simulink model "FMS"  (R2018b)
settings: configuration reference "fms_config" (kept outside this file)
values from neighbouring files (symbols this model uses):
  FMS_EXPORT = Simulink.Parameter(FMS_EXPORT_VALUE)    [fms_model_init.m]
  FMS_PARAM = Simulink.Parameter(FMS_PARAM_VALUE)    [fms_model_init.m]
undefined symbols (not defined in the file or in its folder): actuator_cmd, ax_cmd, ay_cmd, az_cmd, cmd_mask, ControlMode, ctrl_mode, DiscIntNeverNeededParam, FMS_Cmd, FMS_CONST, FMS_Error, home, mode, p_cmd, phi_cmd, PilotMode, psi_rate_cmd, q_cmd, r_cmd, reset, state, status, theta_cmd, throttle_cmd, timestamp, u_cmd, v_cmd, VehicleState, VehicleStatus, w_cmd, wp_consume, wp_current
libraries: simulink x123, FMT_Model_Lib x62, hdlsllib x13
(part 2 of 7)

== system FMS/FMS Commander/Commander/Arm/SubMode/Land ==
  FMS_In : Inport
  Action Port : ActionPort  InitializeStates=reset  ActionType=case
      settings: CopyFcn=Stateflow.SLINSF.SimulinkMan.removeBlockPreDeleteFcn
  Assist Land Speed : Subsystem
  Bus Assignment1 : BusAssignment  AssignedSignals=status,state,ctrl_mode,psi_rate_cmd,u_cmd,v_cmd,w_cmd
  Bus Selector : BusSelector  OutputSignals=Cmd_In.sp_waypoint
  Constant : Constant  Value=0  OutDataTypeStr=Inherit: Inherit via back propagation
  Constant1 : Constant  Value=0  OutDataTypeStr=Bus: FMS_Out_Bus
  Constant2 : Constant  Value=ControlMode.POSCTL
  Constant3 : Constant  Value=VehicleState.Land
  Constant6 : Constant  Value=VehicleStatus.Arm
  Data Type Conversion : DataTypeConversion
  Data Type Conversion1 : DataTypeConversion
  Data Type Conversion2 : DataTypeConversion
  Position Command : Subsystem
  Selector : Selector  InputPortWidth=3  IndexOptions=Index vector (dialog)  Indices=[1 2]  OutputSizes=1
  FMS_Out : Outport
  wires:
  Selector/1 -> Position Command/2(land_xy_R)
  Bus Assignment1/1 -> FMS_Out/1
  Constant1/1 -> Bus Assignment1/1
  Position Command/1(u_cmd_mPs) -> Bus Assignment1/6
  Position Command/2(v_cmd_mPs) -> Bus Assignment1/7
  Constant/1 -> Bus Assignment1/5
  Constant2/1 -> Data Type Conversion2/1
  Constant6/1 -> Data Type Conversion/1
  Data Type Conversion/1 -> Bus Assignment1/2
  Constant3/1 -> Data Type Conversion1/1
  Data Type Conversion1/1 -> Bus Assignment1/3
  Data Type Conversion2/1 -> Bus Assignment1/4
  Bus Selector/1 -> Selector/1  "<sp_waypoint>"
  FMS_In/1 -> Assist Land Speed/1(FMS_In), Position Command/1(FMS_In), Bus Selector/1
  Assist Land Speed/1(w_cmd_mPs) -> Bus Assignment1/8

== system FMS/FMS Commander/Commander/Arm/SubMode/Return ==
  FMS_In : Inport
  Action Port : ActionPort  InitializeStates=reset  ActionType=case
      settings: CopyFcn=Stateflow.SLINSF.SimulinkMan.removeBlockPreDeleteFcn
  Bus Assignment1 : BusAssignment  AssignedSignals=status,state,ctrl_mode,u_cmd,v_cmd,w_cmd,psi_rate_cmd
  Constant1 : Constant  Value=VehicleState.Return
  Constant2 : Constant  Value=0  OutDataTypeStr=Bus: FMS_Out_Bus
  Constant3 : Constant  Value=ControlMode.POSCTL
  Constant6 : Constant  Value=VehicleStatus.Arm
  Data Type Conversion : DataTypeConversion
  Data Type Conversion1 : DataTypeConversion
  Data Type Conversion2 : DataTypeConversion
  Heading Commander : Subsystem
  Sum : Sum  Inputs=+-|
  Velocity Commander : Subsystem
  Way Points : Subsystem
  FMS_Out : Outport
  wires:
  Sum/1 -> Heading Commander/2(p1p2)
  Way Points/2(p2) -> Velocity Commander/2(p2), Sum/1
  Way Points/3(p3) -> Velocity Commander/3(p3)
  Constant3/1 -> Data Type Conversion2/1
  Way Points/1(p1) -> Velocity Commander/1(p1), Sum/2
  Constant2/1 -> Bus Assignment1/1
  Heading Commander/2(psi_rad_cmd) -> Bus Assignment1/8
  Bus Assignment1/1 -> FMS_Out/1
  Data Type Conversion/1 -> Bus Assignment1/2
  Constant6/1 -> Data Type Conversion/1
  Data Type Conversion1/1 -> Bus Assignment1/3
  Data Type Conversion2/1 -> Bus Assignment1/4
  Constant1/1 -> Data Type Conversion1/1
  FMS_In/1 -> Heading Commander/1(FMS_In), Velocity Commander/4(FMS_In), Way Points/1(FMS_In)
  Velocity Commander/1(u_cmd) -> Bus Assignment1/5
  Velocity Commander/2(v_cmd) -> Bus Assignment1/6
  Velocity Commander/3(w_cmd) -> Bus Assignment1/7
  Heading Commander/1(psi_err_rad) -> Velocity Commander/5(psi_err_rad)

== system FMS/FMS Commander/Commander/Arm/SubMode/Takeoff ==
  FMS_In : Inport
  Action Port : ActionPort  InitializeStates=reset  ActionType=case
      settings: CopyFcn=Stateflow.SLINSF.SimulinkMan.removeBlockPreDeleteFcn
  Bus Assignment1 : BusAssignment  AssignedSignals=status,state,ctrl_mode,psi_rate_cmd,u_cmd,v_cmd,w_cmd
  Climb Speed : Subsystem
  Constant : Constant  Value=0  OutDataTypeStr=Inherit: Inherit via back propagation
  Constant1 : Constant  Value=0  OutDataTypeStr=Bus: FMS_Out_Bus
  Constant2 : Constant  Value=ControlMode.POSCTL
  Constant3 : Constant  Value=VehicleState.Takeoff
  Constant5 : Constant  Value=VehicleStatus.Arm
  Data Type Conversion : DataTypeConversion
  Data Type Conversion1 : DataTypeConversion
  Data Type Conversion2 : DataTypeConversion
  Demux : Demux  Outputs=2
  Track Position : Subsystem
  FMS_Out : Outport
  wires:
  Constant5/1 -> Data Type Conversion/1
  Demux/2 -> Bus Assignment1/7
  Demux/1 -> Bus Assignment1/6
  Constant/1 -> Bus Assignment1/5
  Constant2/1 -> Data Type Conversion2/1
  Track Position/1(uv_cmd_mPs) -> Demux/1
  Constant1/1 -> Bus Assignment1/1
  FMS_In/1 -> Climb Speed/1(FMS_In), Track Position/1(FMS_In)
  Bus Assignment1/1 -> FMS_Out/1
  Data Type Conversion/1 -> Bus Assignment1/2
  Data Type Conversion1/1 -> Bus Assignment1/3
  Constant3/1 -> Data Type Conversion1/1
  Data Type Conversion2/1 -> Bus Assignment1/4
  Climb Speed/1(w_cmd_mPs) -> Bus Assignment1/8

== system FMS/FMS Commander/Commander/Arm/SubMode/Unknown ==
  Action Port : ActionPort  InitializeStates=reset  ActionType=default
  Bus Assignment : BusAssignment  AssignedSignals=reset,status,state,actuator_cmd
  Constant : Constant  Value=0  OutDataTypeStr=Bus: FMS_Out_Bus
  Constant1 : Constant  Value=VehicleStatus.Disarm
  Constant2 : Constant  OutDataTypeStr=Inherit: Inherit via back propagation
  Constant3 : Constant  Value=[1000;1000;1000;1000]  VectorParams1D=off  OutDataTypeStr=Inherit: Inherit via back propagation
  Constant4 : Constant  Value=zeros(12,1)  OutDataTypeStr=Inherit: Inherit via back propagation
  Constant5 : Constant  Value=VehicleState.Disarm
  Data Type Conversion : DataTypeConversion
  Data Type Conversion1 : DataTypeConversion
  Mux : Mux  Inputs=2
  FMS_Out : Outport
  wires:
  Mux/1 -> Bus Assignment/5
  Constant4/1 -> Mux/2
  Constant3/1 -> Mux/1
  Constant1/1 -> Data Type Conversion/1
  Constant2/1 -> Bus Assignment/2
  Bus Assignment/1 -> FMS_Out/1
  Constant/1 -> Bus Assignment/1
  Constant5/1 -> Data Type Conversion1/1
  Data Type Conversion/1 -> Bus Assignment/3
  Data Type Conversion1/1 -> Bus Assignment/4

== system FMS/FMS Commander/Commander/Arm/Assist/Acro/Angular Rate Command ==
  FMS_In : Inport
  Bus Selector : BusSelector  OutputSignals=Pilot_Cmd.stick_roll,Pilot_Cmd.stick_pitch,Pilot_Cmd.stick_yaw
  Gain : Gain  Gain=pi  OutDataTypeStr=single
  Gain1 : Gain  Gain=-pi  OutDataTypeStr=single
  Gain2 : Gain  Gain=pi/2  OutDataTypeStr=single
  p_cmd_radPs : Outport
  q_cmd_radPs : Outport  Port=2
  r_cmd_radPs : Outport  Port=3
  wires:
  FMS_In/1 -> Bus Selector/1
  Gain2/1 -> r_cmd_radPs/1
  Gain1/1 -> q_cmd_radPs/1
  Bus Selector/3 -> Gain2/1  "<stick_yaw>"
  Bus Selector/2 -> Gain1/1  "<stick_pitch>"
  Gain/1 -> p_cmd_radPs/1
  Bus Selector/1 -> Gain/1  "<stick_roll>"

== system FMS/FMS Commander/Commander/Arm/Assist/Acro/Throttle Command ==
  FMS_In : Inport
  Add : Sum
  Bus Selector : BusSelector  OutputSignals=Pilot_Cmd.stick_throttle
  Constant4 : Constant  OutDataTypeStr=single
  Constant5 : Constant  Value=1000  OutDataTypeStr=uint16
  Gain2 : Gain  Gain=500  OutDataTypeStr=uint16
  Saturation : Saturate  UpperLimit=2  LowerLimit=0
  Sum : Sum  Inputs=|++
  throttle_cmd : Outport
  wires:
  Constant4/1 -> Sum/2
  Add/1 -> throttle_cmd/1
  Constant5/1 -> Add/2
  Bus Selector/1 -> Sum/1  "<stick_throttle>"
  Saturation/1 -> Gain2/1
  Sum/1 -> Saturation/1
  Gain2/1 -> Add/1
  FMS_In/1 -> Bus Selector/1

== system FMS/FMS Commander/Commander/Arm/Assist/Altitude/Altitude Command ==
  FMS_In : Inport
  Bus Selector : BusSelector  OutputSignals=pilot_cmd_lost
  Constant : Constant  Value=0.5  OutDataTypeStr=single
  Controller : Subsystem
  Detect Movement : Subsystem
  Switch : Switch  Criteria=u2 > Threshold
  w_cmd_mPs : Outport
  wires:
  Controller/1(w_cmd_mPs) -> Switch/3
  Detect Movement/1(motion_state) -> Controller/1(motion_state)
  FMS_In/1 -> Bus Selector/1, Controller/2(FMS_In), Detect Movement/1(FMS_In)
  Bus Selector/1 -> Switch/2  "<pilot_cmd_lost>"
  Constant/1 -> Switch/1
  Switch/1 -> w_cmd_mPs/1

== system FMS/FMS Commander/Commander/Arm/Assist/Altitude/Attitude Command ==
  FMS_In : Inport
  Bus Selector : BusSelector  OutputSignals=Pilot_Cmd.stick_roll,Pilot_Cmd.stick_pitch
  Bus Selector1 : BusSelector  OutputSignals=pilot_cmd_lost
  Compare To Constant : simulink/Logic and Bit Operations/Compare To Constant  relop=>  const=1  OutDataTypeStr=boolean
  Data Type Conversion : DataTypeConversion  OutDataTypeStr=single
  DeadZone : Subsystem  mask{th=FMS_PARAM.MC_ROLL_DZ}
      mask prompts: th "Threshold"
      mask Display: disp('Dead Zone')
  DeadZone2 : Subsystem  mask{th=FMS_PARAM.MC_PITCH_DZ}
      mask prompts: th "Threshold"
      mask Display: disp('Dead Zone')
  Demux : Demux  Outputs=2
  Gain : Gain  Gain=FMS_PARAM.MC_ATT_LIM
  Gain1 : Gain  Gain=-FMS_PARAM.MC_ATT_LIM
  Logical Operator : Logic  Operator=NOT  AllPortsSameDT=off  OutDataTypeStr=boolean
  Multiply : Product
  Multiply1 : Product
  Mux : Mux  Inputs=2
  Phi_CMD_TD : Subsystem
  Switch : Switch  Criteria=u2 > Threshold
  Theta_CMD_TD : Subsystem
  Vector Modulus : FMT_Model_Lib/Math/Vector Modulus
      settings: SourceProductName=FMT Toolbox
  Vector Normalize : FMT_Model_Lib/Math/Vector Normalize
      settings: SourceProductName=FMT Toolbox
  phi_cmd_radPs : Outport
  theta_cmd_radPs : Outport  Port=2
  wires:
  Bus Selector/2 -> DeadZone2/1(u)  "<stick_pitch>"
  Bus Selector/1 -> DeadZone/1(u)  "<stick_roll>"
  FMS_In/1 -> Bus Selector1/1, Bus Selector/1
  Gain/1 -> Multiply/2
  Bus Selector1/1 -> Logical Operator/1  "<pilot_cmd_lost>"
  Multiply/1 -> Phi_CMD_TD/1(v)
  Gain1/1 -> Multiply1/2
  Multiply1/1 -> Theta_CMD_TD/1(v)
  Logical Operator/1 -> Data Type Conversion/1
  Data Type Conversion/1 -> Multiply1/1, Multiply/1
  DeadZone/1(y) -> Mux/1
  DeadZone2/1(y) -> Mux/2
  Mux/1 -> Switch/3, Vector Normalize/1, Vector Modulus/1
  Vector Modulus/1 -> Compare To Constant/1
  Compare To Constant/1 -> Switch/2
  Vector Normalize/1 -> Switch/1
  Switch/1 -> Demux/1
  Demux/1 -> Gain/1
  Demux/2 -> Gain1/1
  Phi_CMD_TD/1(v1) -> phi_cmd_radPs/1
  Theta_CMD_TD/1(v1) -> theta_cmd_radPs/1

== system FMS/FMS Commander/Commander/Arm/Assist/Altitude/Heading Command ==
  FMS_In : Inport
  Controller : Subsystem
  Detect Movement : Subsystem
  psi_rate_cmd_radPs : Outport
  wires:
  FMS_In/1 -> Detect Movement/1(FMS_In), Controller/2(FMS_In)
  Controller/1(psi_rate_cmd_radPs) -> psi_rate_cmd_radPs/1
  Detect Movement/1(motion_state) -> Controller/1(motion_state)

== system FMS/FMS Commander/Commander/Arm/Assist/Position/Altitude Command ==
  FMS_In : Inport
  Bus Selector : BusSelector  OutputSignals=pilot_cmd_lost
  Constant : Constant  Value=0.5  OutDataTypeStr=single
  Controller : Subsystem
  Detect Movement : Subsystem
  Switch : Switch  Criteria=u2 > Threshold
  w_cmd_mPs : Outport
  wires:
  Controller/1(w_cmd_mPs) -> Switch/3
  Detect Movement/1(motion_state) -> Controller/1(motion_state)
  FMS_In/1 -> Bus Selector/1, Controller/2(FMS_In), Detect Movement/1(FMS_In)
  Bus Selector/1 -> Switch/2  "<pilot_cmd_lost>"
  Constant/1 -> Switch/1
  Switch/1 -> w_cmd_mPs/1

== system FMS/FMS Commander/Commander/Arm/Assist/Position/Heading Command ==
  FMS_In : Inport
  Controller : Subsystem
  Detect Movement : Subsystem
  psi_rate_cmd_radPs : Outport
  wires:
  FMS_In/1 -> Detect Movement/1(FMS_In), Controller/2(FMS_In)
  Detect Movement/1(motion_state) -> Controller/1(motion_state)
  Controller/1(psi_rate_cmd_radPs) -> psi_rate_cmd_radPs/1

== system FMS/FMS Commander/Commander/Arm/Assist/Position/Position Command ==
  FMS_In : Inport
  Controller : Subsystem
  Demux : Demux  Outputs=2
  Detect Movement : Subsystem
  u_cmd_mPs : Outport
  v_cmd_mPs : Outport  Port=2
  wires:
  FMS_In/1 -> Controller/2(FMS_In), Detect Movement/1(FMS_In)
  Demux/2 -> v_cmd_mPs/1
  Demux/1 -> u_cmd_mPs/1
  Controller/1(uv_cmd_mPs) -> Demux/1
  Detect Movement/1(motion_state) -> Controller/1(motion_state)

== system FMS/FMS Commander/Commander/Arm/Assist/Stabilize/Attitude Command ==
  FMS_In : Inport
  Bus Selector : BusSelector  OutputSignals=Pilot_Cmd.stick_roll,Pilot_Cmd.stick_pitch
  Bus Selector1 : BusSelector  OutputSignals=pilot_cmd_lost
  Compare To Constant : simulink/Logic and Bit Operations/Compare To Constant  relop=>  const=1  OutDataTypeStr=boolean
  Data Type Conversion : DataTypeConversion  OutDataTypeStr=single
  DeadZone : Subsystem  mask{th=FMS_PARAM.MC_ROLL_DZ}
      mask prompts: th "Threshold"
      mask Display: disp('Dead Zone')
  DeadZone2 : Subsystem  mask{th=FMS_PARAM.MC_PITCH_DZ}
      mask prompts: th "Threshold"
      mask Display: disp('Dead Zone')
  Demux : Demux  Outputs=2
  Gain : Gain  Gain=FMS_PARAM.MC_ATT_LIM
  Gain1 : Gain  Gain=-FMS_PARAM.MC_ATT_LIM
  Logical Operator : Logic  Operator=NOT  AllPortsSameDT=off  OutDataTypeStr=boolean
  Multiply : Product
  Multiply1 : Product
  Mux : Mux  Inputs=2
  Phi_CMD_TD : Subsystem
  Switch : Switch  Criteria=u2 > Threshold
  Theta_CMD_TD : Subsystem
  Vector Modulus : FMT_Model_Lib/Math/Vector Modulus
      settings: SourceProductName=FMT Toolbox
  Vector Normalize : FMT_Model_Lib/Math/Vector Normalize
      settings: SourceProductName=FMT Toolbox
  phi_cmd_radPs : Outport
  theta_cmd_radPs : Outport  Port=2
  wires:
  Bus Selector/2 -> DeadZone2/1(u)  "<stick_pitch>"
  Bus Selector/1 -> DeadZone/1(u)  "<stick_roll>"
  FMS_In/1 -> Bus Selector1/1, Bus Selector/1
  Gain/1 -> Multiply/2
  Bus Selector1/1 -> Logical Operator/1  "<pilot_cmd_lost>"
  Multiply/1 -> Phi_CMD_TD/1(v)
  Gain1/1 -> Multiply1/2
  Multiply1/1 -> Theta_CMD_TD/1(v)
  Logical Operator/1 -> Data Type Conversion/1
  Data Type Conversion/1 -> Multiply1/1, Multiply/1
  DeadZone/1(y) -> Mux/1
  DeadZone2/1(y) -> Mux/2
  Mux/1 -> Switch/3, Vector Normalize/1, Vector Modulus/1
  Vector Modulus/1 -> Compare To Constant/1
  Compare To Constant/1 -> Switch/2
  Vector Normalize/1 -> Switch/1
  Switch/1 -> Demux/1
  Demux/1 -> Gain/1
  Demux/2 -> Gain1/1
  Phi_CMD_TD/1(v1) -> phi_cmd_radPs/1
  Theta_CMD_TD/1(v1) -> theta_cmd_radPs/1

== system FMS/FMS Commander/Commander/Arm/Assist/Stabilize/Heading Command ==
  FMS_In : Inport
  Controller : Subsystem
  Detect Movement : Subsystem
  psi_rate_cmd_radPs : Outport
  wires:
  FMS_In/1 -> Detect Movement/1(FMS_In), Controller/2(FMS_In)
  Controller/1(psi_rate_cmd_radPs) -> psi_rate_cmd_radPs/1
  Detect Movement/1(motion_state) -> Controller/1(motion_state)

== system FMS/FMS Commander/Commander/Arm/Assist/Stabilize/Throttle Command ==
  FMS_In : Inport
  Add : Sum
  Bus Selector : BusSelector  OutputSignals=Pilot_Cmd.stick_throttle
  Bus Selector1 : BusSelector  OutputSignals=pilot_cmd_lost
  Constant : Constant  Value=FMS_PARAM.MC_LAND_LOCK_THRO  OutDataTypeStr=uint16
  Constant4 : Constant  OutDataTypeStr=single
  Constant5 : Constant  Value=1000  OutDataTypeStr=uint16
  Gain2 : Gain  Gain=500  OutDataTypeStr=uint16
  Saturation : Saturate  UpperLimit=2  LowerLimit=0
  Sum : Sum  Inputs=|++
  Switch : Switch  Criteria=u2 > Threshold
  throttle_cmd : Outport
  wires:
  FMS_In/1 -> Bus Selector1/1, Bus Selector/1
  Gain2/1 -> Add/1
  Sum/1 -> Saturation/1
  Saturation/1 -> Gain2/1
  Bus Selector/1 -> Sum/1  "<stick_throttle>"
  Constant5/1 -> Add/2
  Add/1 -> Switch/3
  Constant4/1 -> Sum/2
  Bus Selector1/1 -> Switch/2  "<pilot_cmd_lost>"
  Switch/1 -> throttle_cmd/1
  Constant/1 -> Switch/1

== system FMS/FMS Commander/Commander/Arm/Auto/Mission/Mission_SubSystem ==
  FMS_In : Inport
  Reset : ResetPort  DisableCoverage=on
  Bus Assignment : BusAssignment  AssignedSignals=status,state,ctrl_mode,u_cmd,v_cmd,w_cmd,psi_rate_cmd
  Constant : Constant  Value=0  OutDataTypeStr=Bus: FMS_Out_Bus
  Constant1 : Constant  Value=VehicleStatus.Arm
  Constant2 : Constant  Value=VehicleState.Mission
  Constant3 : Constant  Value=ControlMode.POSCTL
  Data Type Conversion : DataTypeConversion
  Data Type Conversion1 : DataTypeConversion
  Data Type Conversion2 : DataTypeConversion
  Heading Commander : Subsystem
  Velocity Commander : Subsystem
  Way Points : Subsystem
  FMS_Out : Outport
  wires:
  Data Type Conversion1/1 -> Bus Assignment/3
  Way Points/2(p2) -> Velocity Commander/2(p2)
  Constant1/1 -> Data Type Conversion/1
  Heading Commander/2(psi_rad_cmd) -> Bus Assignment/8
  Data Type Conversion2/1 -> Bus Assignment/4
  Data Type Conversion/1 -> Bus Assignment/2
  Constant2/1 -> Data Type Conversion1/1
  Way Points/1(p1) -> Velocity Commander/1(p1)
  Way Points/3(p3) -> Velocity Commander/3(p3)
  Velocity Commander/2(v_cmd) -> Bus Assignment/6
  Heading Commander/1(psi_err_rad) -> Velocity Commander/5(psi_err_rad)
  Constant3/1 -> Data Type Conversion2/1
  Constant/1 -> Bus Assignment/1
  Velocity Commander/3(w_cmd) -> Bus Assignment/7
  FMS_In/1 -> Velocity Commander/4(FMS_In), Heading Commander/1(FMS_In), Way Points/1(FMS_In)
  Velocity Commander/1(u_cmd) -> Bus Assignment/5
  Bus Assignment/1 -> FMS_Out/1

== system FMS/FMS Commander/Commander/Arm/Auto/Offboard/Acc_Command ==
  FMS_In : Inport
  Accel_Command : Subsystem
  Body_FRD : Subsystem
  Bus Selector1 : BusSelector  OutputSignals=INS_Out.psi
  Bus Selector3 : BusSelector  OutputSignals=Auto_Cmd.frame
  Command_Mask : Subsystem
  Demux : Demux  Outputs=3
  Global_Local_NED : Subsystem
  Index Vector : MultiPortSwitch  DataPortOrder=Zero-based contiguous  Inputs=4  zeroidx=on
  Local_FRD : Subsystem
  Multiply : Product
  ax_C_cmd : Outport
  ay_C_cmd : Outport  Port=2
  az_C_cmd : Outport  Port=3
  wires:
  FMS_In/1 -> Bus Selector3/1, Bus Selector1/1, Accel_Command/1(FMS_In), Command_Mask/1(FMS_In)
  Bus Selector3/1 -> Index Vector/1  "<frame>"
  Command_Mask/1(acc_mask) -> Multiply/2
  Global_Local_NED/1(acc_cmd_C) -> Index Vector/3, Index Vector/2
  Local_FRD/1(acc_cmd_C) -> Index Vector/4
  Body_FRD/1(acc_cmd_C) -> Index Vector/5
  Multiply/1 -> Global_Local_NED/2(acc_cmd_O), Body_FRD/1(acc_cmd_B), Local_FRD/2(acc_cmd_R)
  Bus Selector1/1 -> Local_FRD/1(psi), Global_Local_NED/1(psi)  "<psi>"
  Index Vector/1 -> Demux/1
  Demux/1 -> ax_C_cmd/1
  Demux/2 -> ay_C_cmd/1
  Demux/3 -> az_C_cmd/1
  Accel_Command/1(accel_cmd) -> Multiply/1

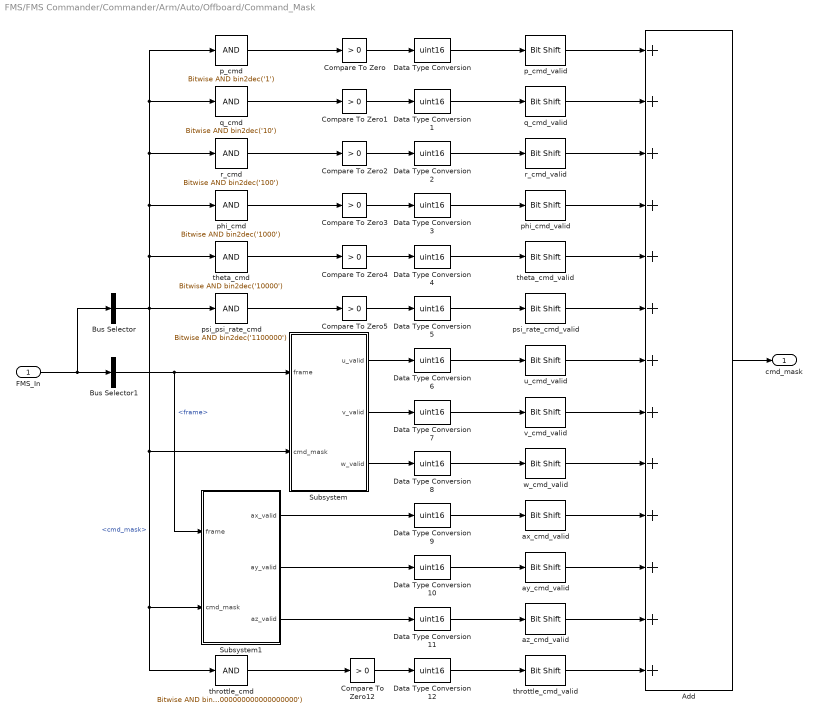
== system FMS/FMS Commander/Commander/Arm/Auto/Offboard/Command_Mask ==
  FMS_In : Inport
  Add : Sum  Inputs=+++++++++++++
  Bus Selector : BusSelector  OutputSignals=Auto_Cmd.cmd_mask
  Bus Selector1 : BusSelector  OutputSignals=Auto_Cmd.frame
  Compare To Zero{,1..5,12} (7 alike) : simulink/Logic and Bit Operations/Compare To Zero  relop=>  OutDataTypeStr=boolean
  Data Type Conversion{,1..12} (13 alike) : DataTypeConversion  OutDataTypeStr=uint16
  Subsystem : Subsystem
  Subsystem1 : Subsystem
  ax_cmd_valid : hdlsllib/Logic and Bit Operations/Bit Shift  mode=Shift Left Logical  N=9
      settings: SourceProductName=HDL Coder  SourceProductBaseCode=HD
  ay_cmd_valid : hdlsllib/Logic and Bit Operations/Bit Shift  mode=Shift Left Logical  N=10
      settings: SourceProductName=HDL Coder  SourceProductBaseCode=HD
  az_cmd_valid : hdlsllib/Logic and Bit Operations/Bit Shift  mode=Shift Left Logical  N=11
      settings: SourceProductName=HDL Coder  SourceProductBaseCode=HD
  p_cmd : simulink/Logic and Bit Operations/Bitwise Operator  logicop=AND  UseBitMask=on  BitMask=bin2dec('1')  BitMaskRealWorld=Stored Integer
  p_cmd_valid : hdlsllib/Logic and Bit Operations/Bit Shift  mode=Shift Left Logical  N=0
      settings: SourceProductName=HDL Coder  SourceProductBaseCode=HD
  phi_cmd : simulink/Logic and Bit Operations/Bitwise Operator  logicop=AND  UseBitMask=on  BitMask=bin2dec('1000')  BitMaskRealWorld=Stored Integer
  phi_cmd_valid : hdlsllib/Logic and Bit Operations/Bit Shift  mode=Shift Left Logical  N=3
      settings: SourceProductName=HDL Coder  SourceProductBaseCode=HD
  psi_psi_rate_cmd : simulink/Logic and Bit Operations/Bitwise Operator  logicop=AND  UseBitMask=on  BitMask=bin2dec('1100000')  BitMaskRealWorld=Stored Integer
  psi_rate_cmd_valid : hdlsllib/Logic and Bit Operations/Bit Shift  mode=Shift Left Logical  N=5
      settings: SourceProductName=HDL Coder  SourceProductBaseCode=HD
  q_cmd : simulink/Logic and Bit Operations/Bitwise Operator  logicop=AND  UseBitMask=on  BitMask=bin2dec('10')  BitMaskRealWorld=Stored Integer
  q_cmd_valid : hdlsllib/Logic and Bit Operations/Bit Shift  mode=Shift Left Logical  N=1
      settings: SourceProductName=HDL Coder  SourceProductBaseCode=HD
  r_cmd : simulink/Logic and Bit Operations/Bitwise Operator  logicop=AND  UseBitMask=on  BitMask=bin2dec('100')  BitMaskRealWorld=Stored Integer
  r_cmd_valid : hdlsllib/Logic and Bit Operations/Bit Shift  mode=Shift Left Logical  N=2
      settings: SourceProductName=HDL Coder  SourceProductBaseCode=HD
  theta_cmd : simulink/Logic and Bit Operations/Bitwise Operator  logicop=AND  UseBitMask=on  BitMask=bin2dec('10000')  BitMaskRealWorld=Stored Integer
  theta_cmd_valid : hdlsllib/Logic and Bit Operations/Bit Shift  mode=Shift Left Logical  N=4
      settings: SourceProductName=HDL Coder  SourceProductBaseCode=HD
  throttle_cmd : simulink/Logic and Bit Operations/Bitwise Operator  logicop=AND  UseBitMask=on  BitMask=bin2dec('10000000000000000000')  BitMaskRealWorld=Stored Integer
  throttle_cmd_valid : hdlsllib/Logic and Bit Operations/Bit Shift  mode=Shift Left Logical  N=12
      settings: SourceProductName=HDL Coder  SourceProductBaseCode=HD
  u_cmd_valid : hdlsllib/Logic and Bit Operations/Bit Shift  mode=Shift Left Logical  N=6
      settings: SourceProductName=HDL Coder  SourceProductBaseCode=HD
  v_cmd_valid : hdlsllib/Logic and Bit Operations/Bit Shift  mode=Shift Left Logical  N=7
      settings: SourceProductName=HDL Coder  SourceProductBaseCode=HD
  w_cmd_valid : hdlsllib/Logic and Bit Operations/Bit Shift  mode=Shift Left Logical  N=8
      settings: SourceProductName=HDL Coder  SourceProductBaseCode=HD
  cmd_mask : Outport
  wires:
  FMS_In/1 -> Bus Selector/1, Bus Selector1/1
  p_cmd/1 -> Compare To Zero/1
  Compare To Zero/1 -> Data Type Conversion/1
  Data Type Conversion/1 -> p_cmd_valid/1
  q_cmd/1 -> Compare To Zero1/1
  Compare To Zero1/1 -> Data Type Conversion1/1
  Data Type Conversion1/1 -> q_cmd_valid/1
  r_cmd/1 -> Compare To Zero2/1
  Compare To Zero2/1 -> Data Type Conversion2/1
  Data Type Conversion2/1 -> r_cmd_valid/1
  Data Type Conversion3/1 -> phi_cmd_valid/1
  phi_cmd/1 -> Compare To Zero3/1
  Compare To Zero3/1 -> Data Type Conversion3/1
  Data Type Conversion4/1 -> theta_cmd_valid/1
  theta_cmd/1 -> Compare To Zero4/1
  Compare To Zero4/1 -> Data Type Conversion4/1
  psi_psi_rate_cmd/1 -> Compare To Zero5/1
  Compare To Zero5/1 -> Data Type Conversion5/1
  Data Type Conversion5/1 -> psi_rate_cmd_valid/1
  Data Type Conversion9/1 -> ax_cmd_valid/1
  Bus Selector/1 -> q_cmd/1, p_cmd/1, r_cmd/1, phi_cmd/1, theta_cmd/1, throttle_cmd/1, Subsystem1/2(cmd_mask), Subsystem/2(cmd_mask), psi_psi_rate_cmd/1  "<cmd_mask>"
  Data Type Conversion10/1 -> ay_cmd_valid/1
  Data Type Conversion11/1 -> az_cmd_valid/1
  throttle_cmd/1 -> Compare To Zero12/1
  Compare To Zero12/1 -> Data Type Conversion12/1
  Data Type Conversion12/1 -> throttle_cmd_valid/1
  p_cmd_valid/1 -> Add/1
  q_cmd_valid/1 -> Add/2
  r_cmd_valid/1 -> Add/3
  phi_cmd_valid/1 -> Add/4
  theta_cmd_valid/1 -> Add/5
  psi_rate_cmd_valid/1 -> Add/6
  ax_cmd_valid/1 -> Add/10
  ay_cmd_valid/1 -> Add/11
  az_cmd_valid/1 -> Add/12
  throttle_cmd_valid/1 -> Add/13
  Add/1 -> cmd_mask/1
  u_cmd_valid/1 -> Add/7
  v_cmd_valid/1 -> Add/8
  w_cmd_valid/1 -> Add/9
  Data Type Conversion7/1 -> v_cmd_valid/1
  Data Type Conversion8/1 -> w_cmd_valid/1
  Data Type Conversion6/1 -> u_cmd_valid/1
  Subsystem/1(u_valid) -> Data Type Conversion6/1
  Subsystem/2(v_valid) -> Data Type Conversion7/1
  Subsystem/3(w_valid) -> Data Type Conversion8/1
  Bus Selector1/1 -> Subsystem/1(frame), Subsystem1/1(frame)  "<frame>"
  Subsystem1/1(ax_valid) -> Data Type Conversion9/1
  Subsystem1/2(ay_valid) -> Data Type Conversion10/1
  Subsystem1/3(az_valid) -> Data Type Conversion11/1

== system FMS/FMS Commander/Commander/Arm/Auto/Offboard/Heading_Command ==
  FMS_In : Inport
  Heading_Control : Subsystem
  Psi_Rate_Command : Subsystem
  Saturation : Saturate  UpperLimit=FMS_PARAM.MC_YAWRATE_LIM  LowerLimit=-FMS_PARAM.MC_YAWRATE_LIM
  Sum : Sum  Inputs=|++
  psi_rate_cmd : Outport
  wires:
  Sum/1 -> Saturation/1
  FMS_In/1 -> Heading_Control/1(FMS_In), Psi_Rate_Command/1(FMS_In)
  Heading_Control/1(psi_rate_cmd) -> Sum/1
  Psi_Rate_Command/1(psi_rate_cmd) -> Sum/2
  Saturation/1 -> psi_rate_cmd/1

== system FMS/FMS Commander/Commander/Arm/Auto/Offboard/Velocity_Command ==
  FMS_In : Inport
  Demux : Demux  Outputs=3
  Position_Control : Subsystem
  Saturation1 : Saturate  UpperLimit=FMS_PARAM.MC_VEL_XY_LIM  LowerLimit=-FMS_PARAM.MC_VEL_XY_LIM
  Saturation2 : Saturate  UpperLimit=FMS_PARAM.MC_VEL_XY_LIM  LowerLimit=-FMS_PARAM.MC_VEL_XY_LIM
  Saturation3 : Saturate  UpperLimit=FMS_PARAM.MC_VEL_Z_LIM  LowerLimit=-FMS_PARAM.MC_VEL_Z_LIM
  Sum1 : Sum  Inputs=|++
  Velocity_Command : Subsystem
  u_cmd : Outport
  v_cmd : Outport  Port=2
  w_cmd : Outport  Port=3
  wires:
  FMS_In/1 -> Velocity_Command/1(FMS_In), Position_Control/1(FMS_In)
  Position_Control/1(vel_cmd_C) -> Sum1/1
  Velocity_Command/1(vel_cmd_C) -> Sum1/2
  Demux/1 -> Saturation2/1
  Demux/2 -> Saturation1/1
  Demux/3 -> Saturation3/1
  Sum1/1 -> Demux/1
  Saturation2/1 -> u_cmd/1
  Saturation1/1 -> v_cmd/1
  Saturation3/1 -> w_cmd/1

== system FMS/FMS Commander/Commander/Arm/SubMode/Hold/Altitude Hold ==
  FMS_In : Inport
  Controller : Subsystem
  Detect Movement : Subsystem
  w_cmd_mPs : Outport
  wires:
  Controller/1(w_cmd_mPs) -> w_cmd_mPs/1
  Detect Movement/1(motion_state) -> Controller/1(motion_state)
  FMS_In/1 -> Controller/2(FMS_In), Detect Movement/1(FMS_In)

== system FMS/FMS Commander/Commander/Arm/SubMode/Hold/Heading Hold ==
  FMS_In : Inport
  Controller : Subsystem
  Detect Movement : Subsystem
  psi_rate_cmd_radPs : Outport
  wires:
  Controller/1(psi_rate_cmd_radPs) -> psi_rate_cmd_radPs/1
  Detect Movement/1(motion_state) -> Controller/1(motion_state)
  FMS_In/1 -> Controller/2(FMS_In), Detect Movement/1(FMS_In)

== system FMS/FMS Commander/Commander/Arm/SubMode/Hold/Position Hold ==
  FMS_In : Inport
  Controller : Subsystem
  Demux : Demux  Outputs=2
  Detect Movement : Subsystem
  u_cmd_mPs : Outport
  v_cmd_mPs : Outport  Port=2
  wires:
  FMS_In/1 -> Controller/2(FMS_In), Detect Movement/1(FMS_In)
  Demux/2 -> v_cmd_mPs/1
  Demux/1 -> u_cmd_mPs/1
  Controller/1(uv_cmd_mPs) -> Demux/1
  Detect Movement/1(motion_state) -> Controller/1(motion_state)

== system FMS/FMS Commander/Commander/Arm/SubMode/Land/Assist Land Speed ==
  FMS_In : Inport
  Bus Selector1 : BusSelector  OutputSignals=INS_Out.flag,INS_Out.h_AGL
  Compare To Constant : simulink/Logic and Bit Operations/Compare To Constant  relop=<=  const=FMS_PARAM.MC_ASSIST_LAND_H  OutDataTypeStr=boolean
  Gain : Gain  Gain=0.5
  Land_Speed : Constant  Value=FMS_PARAM.MC_LAND_SPEED  OutDataTypeStr=Inherit: Inherit via back propagation
  Logical Operator : Logic  AllPortsSameDT=off  OutDataTypeStr=boolean
  Switch : Switch  Criteria=u2 > Threshold
  TD : Subsystem
  cmd_p valid : simulink/Logic and Bit Operations/Bitwise Operator  logicop=AND  UseBitMask=on  BitMask=bin2dec('100000000')  BitMaskRealWorld=Stored Integer
  w_cmd_mPs : Outport
  wires:
  Land_Speed/1 -> Switch/3, Gain/1
  Gain/1 -> Switch/1
  Compare To Constant/1 -> Logical Operator/2
  FMS_In/1 -> Bus Selector1/1
  cmd_p valid/1 -> Logical Operator/1  "h_AGL_valid"
  Bus Selector1/1 -> cmd_p valid/1  "<flag>"
  Bus Selector1/2 -> Compare To Constant/1  "<h_AGL>"
  Logical Operator/1 -> Switch/2
  Switch/1 -> TD/1(v)
  TD/1(v1) -> w_cmd_mPs/1

== system FMS/FMS Commander/Commander/Arm/SubMode/Land/Position Command ==
  FMS_In : Inport
  land_xy_R : Inport  Port=2
  Demux : Demux  Outputs=2
  Position Control : Subsystem
  Saturation1 : Saturate  UpperLimit=FMS_PARAM.MC_VEL_XY_LIM/5  LowerLimit=-FMS_PARAM.MC_VEL_XY_LIM/5
  u_cmd_mPs : Outport
  v_cmd_mPs : Outport  Port=2
  wires:
  land_xy_R/1 -> Position Control/2(land_xy_R)
  Position Control/1(uv_cmd_mPs) -> Saturation1/1
  Demux/2 -> v_cmd_mPs/1
  Demux/1 -> u_cmd_mPs/1
  Saturation1/1 -> Demux/1
  FMS_In/1 -> Position Control/1(FMS_In)

== system FMS/FMS Commander/Commander/Arm/SubMode/Return/Heading Commander ==
  FMS_In : Inport
  p1p2 : Inport  Port=2
  Heading Control : Subsystem
  Included Angle : Subsystem
  North : Constant  Value=[1 0]  OutDataTypeStr=single
  psi_err_rad : Outport
  psi_rad_cmd : Outport  Port=2
  wires:
  p1p2/1 -> Included Angle/2(vec2)
  FMS_In/1 -> Heading Control/1(FMS_In)
  North/1 -> Included Angle/1(vec1)
  Included Angle/1(angle_rad) -> Heading Control/2(psi_cmd_rad)
  Heading Control/1(psi_rate_cmd_radPs) -> psi_rad_cmd/1
  Heading Control/2(psi_err_rad) -> psi_err_rad/1

== system FMS/FMS Commander/Commander/Arm/SubMode/Return/Velocity Commander ==
  p1 : Inport
  p2 : Inport  Port=2
  p3 : Inport  Port=3
  In Bus Element3 : Inport  Port=4  PortName=FMS_In
  In Bus Element4 : Inport  Port=4  PortName=FMS_In
  In Bus Element : Inport  Port=4  PortName=FMS_In  Element=INS_Out.vn
  In Bus Element1 : Inport  Port=4  PortName=FMS_In  Element=INS_Out.ve
  In Bus Element2 : Inport  Port=4  PortName=FMS_In  Element=INS_Out.psi
  In Bus Element5 : Inport  Port=4  PortName=FMS_In  Element=Cmd_In.set_speed
  psi_err_rad : Inport  Port=5
  Abs : Abs
  Altitude Control : Subsystem
  Compare To Constant : simulink/Logic and Bit Operations/Compare To Constant  relop=<=  const=10/180*pi  OutDataTypeStr=boolean
  Compare To Zero : simulink/Logic and Bit Operations/Compare To Zero  relop===  OutDataTypeStr=boolean
  Cruise Speed : Subsystem
  Demux : Demux  Outputs=3
  Gain : Gain  Gain=FMS_PARAM.MC_L1_GAIN  OutDataTypeStr=single
  Hold Position : Subsystem
  L1 Reference WP : Subsystem
  Lateral Acceleration : Subsystem
  Lateral Acceleration To Speed : Subsystem
  Mux1 : Mux  Inputs=2
  Switch : Switch  Criteria=u2 > Threshold
  "Target Speed " : Subsystem
  ValidCounter : Subsystem
  u_cmd : Outport
  v_cmd : Outport  Port=2
  w_cmd : Outport  Port=3
  wires:
  p3/1 -> "Target Speed "/1(P3), Lateral Acceleration To Speed/2(p3), Lateral Acceleration/3(p3), L1 Reference WP/3(P3)
  In Bus Element1/1 -> Mux1/2
  Mux1/1 -> Lateral Acceleration/1(Vg)
  p2/1 -> "Target Speed "/2(P2), Lateral Acceleration To Speed/3(p2), L1 Reference WP/2(P2)
  Demux/2 -> v_cmd/1
  Demux/3 -> w_cmd/1
  Demux/1 -> u_cmd/1
  In Bus Element/1 -> Mux1/1
  L1 Reference WP/1(L1_WP) -> Lateral Acceleration/2(L1_WP)  "L1_WP"
  p1/1 -> L1 Reference WP/1(P1)
  Lateral Acceleration/1(l1_a_cmd) -> Lateral Acceleration To Speed/1(l1_a)  "l1_a_cmd"
  In Bus Element2/1 -> Lateral Acceleration To Speed/4(psi)
  "Target Speed "/1(Vg) -> Lateral Acceleration To Speed/5(Vg)  "Vg"
  Lateral Acceleration To Speed/1(Vg_C_cmd) -> Altitude Control/2(Vg_C_cmd)
  psi_err_rad/1 -> Abs/1
  Abs/1 -> Compare To Constant/1
  In Bus Element3/1 -> Hold Position/1(FMS_In)
  Hold Position/1(vel_cmd) -> Switch/1
  Switch/1 -> Demux/1
  Altitude Control/1(vel_C_cmd) -> Switch/3
  In Bus Element4/1 -> Altitude Control/1(FMS_In)
  Compare To Constant/1 -> ValidCounter/1(in)
  ValidCounter/1(out) -> Compare To Zero/1
  Compare To Zero/1 -> Lateral Acceleration To Speed/7(rotating), "Target Speed "/4(rotating), Switch/2
  Cruise Speed/1(cruise_speed) -> Gain/1, Lateral Acceleration To Speed/6(cruise_speed), "Target Speed "/3(cruise_speed)
  In Bus Element5/1 -> Cruise Speed/1(config_speed)
  Gain/1 -> L1 Reference WP/4(L1), Lateral Acceleration/4(L1)

== system FMS/FMS Commander/Commander/Arm/SubMode/Return/Way Points ==
  note: P1: path start point
      | P2: path end point
      | P3: vehicle point
  FMS_In : Inport
  Bus Selector : BusSelector  OutputSignals=INS_Out.x_R,INS_Out.y_R
  Bus Selector1 : BusSelector  OutputSignals=Cmd_In.sp_waypoint
  Delay : Delay  DelayLength=1  InitialConditionSource=Input port  InitialCondition=single([0 0])
      settings: InputPortMap=u0,p4
  Mux : Mux  Inputs=2
  Reshape : Reshape  OutputDimensionality=Customize  OutputDimensions=[2,1]
  Reshape1 : Reshape  OutputDimensionality=Customize  OutputDimensions=[2,1]
  Reshape2 : Reshape  OutputDimensionality=Customize  OutputDimensions=[2,1]
  Selector : Selector  InputPortWidth=3  IndexOptions=Index vector (dialog)  Indices=[1 2]  OutputSizes=1
  p1 : Outport
  p2 : Outport  Port=2
  p3 : Outport  Port=3
  wires:
  Reshape2/1 -> p3/1
  Reshape1/1 -> p1/1
  Reshape/1 -> p2/1
  Bus Selector/2 -> Mux/2  "<y_R>"
  Bus Selector/1 -> Mux/1  "<x_R>"
  Mux/1 -> Reshape2/1, Delay/2
  Delay/1 -> Delay/1, Reshape1/1
  FMS_In/1 -> Bus Selector1/1, Bus Selector/1
  Bus Selector1/1 -> Selector/1  "<sp_waypoint>"
  Selector/1 -> Reshape/1

== system FMS/FMS Commander/Commander/Arm/SubMode/Takeoff/Climb Speed ==
  FMS_In : Inport
  Abs : Abs
  Abs1 : Abs
  Bus Selector : BusSelector  OutputSignals=INS_Out.h_R
  Bus Selector1 : BusSelector  OutputSignals=Cmd_In.cur_waypoint
  Bus Selector2 : BusSelector  OutputSignals=Cmd_In.sp_waypoint
  Compare To Constant : simulink/Logic and Bit Operations/Compare To Constant  relop=>  const=2.0  OutDataTypeStr=boolean
  Compare To Constant1 : simulink/Logic and Bit Operations/Compare To Constant  relop=>  const=2.0  OutDataTypeStr=boolean
  Gain : Gain  Gain=0.5
  Logical Operator : Logic  AllPortsSameDT=off  OutDataTypeStr=boolean
  Selector : Selector  InputPortWidth=3  IndexOptions=Index vector (dialog)  Indices=3  OutputSizes=1
  Selector1 : Selector  InputPortWidth=3  IndexOptions=Index vector (dialog)  Indices=3  OutputSizes=1
  Sum : Sum  Inputs=|+-
  Sum1 : Sum  Inputs=|+-
  Switch : Switch  Criteria=u2 ~= 0  Threshold=2
  TD : Subsystem
  Takeoff_Speed : Constant  Value=-FMS_PARAM.MC_TAKEOFF_SPEED  OutDataTypeStr=Inherit: Inherit via back propagation
  w_cmd_mPs : Outport
  wires:
  Takeoff_Speed/1 -> Gain/1, Switch/1
  Sum/1 -> Abs/1
  Bus Selector/1 -> Sum1/2, Sum/1  "<h_R>"
  Switch/1 -> TD/1(v)
  FMS_In/1 -> Bus Selector2/1, Bus Selector/1, Bus Selector1/1
  Selector/1 -> Sum/2
  Bus Selector1/1 -> Selector/1  "<cur_waypoint>"
  Abs/1 -> Compare To Constant1/1
  Bus Selector2/1 -> Selector1/1  "<sp_waypoint>"
  Selector1/1 -> Sum1/1
  Sum1/1 -> Abs1/1
  Abs1/1 -> Compare To Constant/1
  Compare To Constant/1 -> Logical Operator/1
  Compare To Constant1/1 -> Logical Operator/2
  Logical Operator/1 -> Switch/2
  TD/1(v1) -> w_cmd_mPs/1
  Gain/1 -> Switch/3

== system FMS/FMS Commander/Commander/Arm/SubMode/Takeoff/Track Position ==
  FMS_In : Inport
  Bus Selector : BusSelector  OutputSignals=INS_Out.psi
  Bus_Selection : Subsystem
  Constant : Constant  Value=0  OutDataTypeStr=Inherit: Inherit via back propagation
  Gain2 : Gain  Gain=FMS_PARAM.MC_XY_P  OutDataTypeStr=single
  Multiply : Product  Multiplication=Matrix(*)
  Mux : Mux  Inputs=2
  Psi To DCM : FMT_Model_Lib/Transformation/Psi To DCM
      settings: SourceProductName=FMT Toolbox
  Saturation1 : Saturate  UpperLimit=FMS_PARAM.MC_VEL_XY_LIM/5  LowerLimit=-FMS_PARAM.MC_VEL_XY_LIM/5
  Selector : Selector  InputPortWidth=3  IndexOptions=Index vector (dialog)  Indices=[1 2]  OutputSizes=1
  Sum : Sum  Inputs=-+|
  Target Position : Subsystem
  uv_cmd_mPs : Outport
  wires:
  Saturation1/1 -> uv_cmd_mPs/1
  Bus Selector/1 -> Psi To DCM/1  "<psi>"
  Selector/1 -> Gain2/1
  Mux/1 -> Multiply/2
  Multiply/1 -> Selector/1
  Psi To DCM/1 -> Multiply/1  "M_CO"
  Constant/1 -> Mux/2
  FMS_In/1 -> Bus Selector/1, Target Position/1(FMS_In), Bus_Selection/1(FMS_In)
  Sum/1 -> Mux/1  "xy_err_R"
  Bus_Selection/1(xy_est_R) -> Sum/1  "xy_est_R"
  Gain2/1 -> Saturation1/1
  Target Position/1(xy_cmd_R) -> Sum/2

== system FMS/FMS Commander/Commander/Arm/Assist/Altitude/Altitude Command/Controller ==
  motion_state : Inport
  In Bus Element : Inport  Port=2  PortName=FMS_In
  In Bus Element1 : Inport  Port=2  PortName=FMS_In
  Hold Control : Subsystem  TreatAsAtomicUnit=on
  Merge : Merge
  Move Control : Subsystem  TreatAsAtomicUnit=on
  Saturation1 : Saturate  UpperLimit=FMS_PARAM.MC_VEL_Z_LIM  LowerLimit=-FMS_PARAM.MC_VEL_Z_LIM
  Switch Case : SwitchCase  CaseConditions={MotionState.Hold, [MotionState.Brake, MotionState.Move]}  ShowDefaultCase=off
  w_cmd_mPs : Outport
  wires:
  Move Control/1(w_cmd_mPs) -> Merge/2
  Hold Control/1(w_cmd_mPs) -> Merge/1
  In Bus Element/1 -> Hold Control/1(FMS_In)
  Switch Case/1 -> Hold Control/Action
  motion_state/1 -> Switch Case/1
  Saturation1/1 -> w_cmd_mPs/1
  Merge/1 -> Saturation1/1
  Switch Case/2 -> Move Control/Action
  In Bus Element1/1 -> Move Control/1(FMS_In)

== system FMS/FMS Commander/Commander/Arm/Assist/Altitude/Altitude Command/Detect Movement ==
  FMS_In : Inport
  Abs : Abs
  Abs1 : Abs
  Bus Selector : BusSelector  OutputSignals=Pilot_Cmd.stick_throttle,INS_Out.vd
  Compare To Constant : simulink/Logic and Bit Operations/Compare To Constant  relop=>  const=FMS_PARAM.MC_THROTTLE_DZ  OutDataTypeStr=boolean
  Motion Status : Stateflow chart  TreatAsAtomicUnit=on
  motion_state : Outport
  wires:
  FMS_In/1 -> Bus Selector/1
  Abs1/1 -> Compare To Constant/1
  Motion Status/1(state) -> motion_state/1
  Compare To Constant/1 -> Motion Status/1(motion_req)
  Abs/1 -> Motion Status/2(speed)
  Bus Selector/1 -> Abs1/1  "<stick_throttle>"
  Bus Selector/2 -> Abs/1  "<vd>"

== system FMS/FMS Commander/Commander/Arm/Assist/Altitude/Attitude Command/DeadZone ==
  u : Inport
  Dead Zone : DeadZone  LowerValue=-th  UpperValue=th  SaturateOnIntegerOverflow=on
  Gain : Gain  Gain=1/(1-th)
  y : Outport
  wires:
  Gain/1 -> y/1
  Dead Zone/1 -> Gain/1
  u/1 -> Dead Zone/1

== system FMS/FMS Commander/Commander/Arm/Assist/Altitude/Attitude Command/DeadZone2 ==
  u : Inport
  Dead Zone : DeadZone  LowerValue=-th  UpperValue=th  SaturateOnIntegerOverflow=on
  Gain : Gain  Gain=1/(1-th)
  y : Outport
  wires:
  u/1 -> Dead Zone/1
  Dead Zone/1 -> Gain/1
  Gain/1 -> y/1

== system FMS/FMS Commander/Commander/Arm/Assist/Altitude/Attitude Command/Phi_CMD_TD ==
  v : Inport
  Constant : Constant  Value=FMS_PARAM.MC_STICK_SENS
  Integrator : DiscreteIntegrator  SampleTime=-1  ICPrevOutput=DiscIntNeverNeededParam  ICPrevScaledInput=DiscIntNeverNeededParam
  Integrator1 : DiscreteIntegrator  SampleTime=-1  ICPrevOutput=DiscIntNeverNeededParam  ICPrevScaledInput=DiscIntNeverNeededParam
  Subtract : Sum  Inputs=+-
  "fhan " : Subsystem  mask{r0=10*pi, h0=0.04}
      mask DialogControl ParameterGroupVar Prompt: fhan(v1,v2,r0,h0)
  v1 : Outport
  wires:
  "fhan "/1(fhan) -> Integrator/1
  Subtract/1 -> "fhan "/1(v1)
  Integrator/1 -> Integrator1/1, "fhan "/2(v2)  "v2"
  v/1 -> Subtract/2
  Integrator1/1 -> Subtract/1, v1/1
  Constant/1 -> "fhan "/3(scale)

== system FMS/FMS Commander/Commander/Arm/Assist/Altitude/Attitude Command/Theta_CMD_TD ==
  v : Inport
  Constant : Constant  Value=FMS_PARAM.MC_STICK_SENS
  Integrator : DiscreteIntegrator  SampleTime=-1  ICPrevOutput=DiscIntNeverNeededParam  ICPrevScaledInput=DiscIntNeverNeededParam
  Integrator1 : DiscreteIntegrator  SampleTime=-1  ICPrevOutput=DiscIntNeverNeededParam  ICPrevScaledInput=DiscIntNeverNeededParam
  Subtract : Sum  Inputs=+-
  "fhan " : Subsystem  mask{r0=10*pi, h0=0.04}
      mask DialogControl ParameterGroupVar Prompt: fhan(v1,v2,r0,h0)
  v1 : Outport
  wires:
  Integrator1/1 -> v1/1, Subtract/1
  v/1 -> Subtract/2
  Integrator/1 -> Integrator1/1, "fhan "/2(v2)  "v2"
  Subtract/1 -> "fhan "/1(v1)
  "fhan "/1(fhan) -> Integrator/1
  Constant/1 -> "fhan "/3(scale)

== system FMS/FMS Commander/Commander/Arm/Assist/Altitude/Heading Command/Controller ==
  motion_state : Inport
  In Bus Element : Inport  Port=2  PortName=FMS_In
  In Bus Element1 : Inport  Port=2  PortName=FMS_In
  Hold Control : Subsystem  TreatAsAtomicUnit=on
  Merge : Merge
  Move Control : Subsystem  TreatAsAtomicUnit=on
  Saturation : Saturate  UpperLimit=FMS_PARAM.MC_YAWRATE_LIM  LowerLimit=-FMS_PARAM.MC_YAWRATE_LIM
  Switch Case : SwitchCase  CaseConditions={MotionState.Hold, [MotionState.Brake, MotionState.Move]}  ShowDefaultCase=off
  psi_rate_cmd_radPs : Outport
  wires:
  Move Control/1(psi_rate_cmd_radPs) -> Merge/2
  Hold Control/1(psi_rate_cmd_radPs) -> Merge/1
  In Bus Element/1 -> Hold Control/1(FMS_In)
  Switch Case/2 -> Move Control/Action
  Switch Case/1 -> Hold Control/Action
  motion_state/1 -> Switch Case/1
  Saturation/1 -> psi_rate_cmd_radPs/1
  Merge/1 -> Saturation/1
  In Bus Element1/1 -> Move Control/1(FMS_In)

== system FMS/FMS Commander/Commander/Arm/Assist/Altitude/Heading Command/Detect Movement ==
  FMS_In : Inport
  Abs : Abs
  Abs1 : Abs
  Bus Selector : BusSelector  OutputSignals=Pilot_Cmd.stick_yaw,INS_Out.r
  Compare To Constant : simulink/Logic and Bit Operations/Compare To Constant  relop=>  const=FMS_PARAM.MC_YAW_DZ  OutDataTypeStr=boolean
  Motion State : Stateflow chart  TreatAsAtomicUnit=on
  motion_state : Outport
  wires:
  FMS_In/1 -> Bus Selector/1
  Abs1/1 -> Compare To Constant/1
  Motion State/1(state) -> motion_state/1
  Compare To Constant/1 -> Motion State/1(motion_req)
  Abs/1 -> Motion State/2(speed)
  Bus Selector/1 -> Abs1/1  "<stick_yaw>"
  Bus Selector/2 -> Abs/1  "<r>"

== system FMS/FMS Commander/Commander/Arm/Assist/Position/Altitude Command/Controller ==
  motion_state : Inport
  In Bus Element : Inport  Port=2  PortName=FMS_In
  In Bus Element1 : Inport  Port=2  PortName=FMS_In
  Hold Control : Subsystem  TreatAsAtomicUnit=on
  Merge : Merge
  Move Control : Subsystem  TreatAsAtomicUnit=on
  Saturation1 : Saturate  UpperLimit=FMS_PARAM.MC_VEL_Z_LIM  LowerLimit=-FMS_PARAM.MC_VEL_Z_LIM
  Switch Case : SwitchCase  CaseConditions={MotionState.Hold, [MotionState.Brake, MotionState.Move]}  ShowDefaultCase=off
  w_cmd_mPs : Outport
  wires:
  Move Control/1(w_cmd_mPs) -> Merge/2
  Hold Control/1(w_cmd_mPs) -> Merge/1
  In Bus Element/1 -> Hold Control/1(FMS_In)
  Switch Case/1 -> Hold Control/Action
  motion_state/1 -> Switch Case/1
  Saturation1/1 -> w_cmd_mPs/1
  Merge/1 -> Saturation1/1
  Switch Case/2 -> Move Control/Action
  In Bus Element1/1 -> Move Control/1(FMS_In)

== system FMS/FMS Commander/Commander/Arm/Assist/Position/Altitude Command/Detect Movement ==
  FMS_In : Inport
  Abs : Abs
  Abs1 : Abs
  Bus Selector : BusSelector  OutputSignals=Pilot_Cmd.stick_throttle,INS_Out.vd
  Compare To Constant : simulink/Logic and Bit Operations/Compare To Constant  relop=>  const=FMS_PARAM.MC_THROTTLE_DZ  OutDataTypeStr=boolean
  Motion Status : Stateflow chart  TreatAsAtomicUnit=on
  motion_state : Outport
  wires:
  FMS_In/1 -> Bus Selector/1
  Abs1/1 -> Compare To Constant/1
  Motion Status/1(state) -> motion_state/1
  Compare To Constant/1 -> Motion Status/1(motion_req)
  Abs/1 -> Motion Status/2(speed)
  Bus Selector/1 -> Abs1/1  "<stick_throttle>"
  Bus Selector/2 -> Abs/1  "<vd>"

== system FMS/FMS Commander/Commander/Arm/Assist/Position/Heading Command/Controller ==
  motion_state : Inport
  In Bus Element : Inport  Port=2  PortName=FMS_In
  In Bus Element1 : Inport  Port=2  PortName=FMS_In
  Hold Control : Subsystem  TreatAsAtomicUnit=on
  Merge : Merge
  Move Control : Subsystem  TreatAsAtomicUnit=on
  Saturation : Saturate  UpperLimit=FMS_PARAM.MC_YAWRATE_LIM  LowerLimit=-FMS_PARAM.MC_YAWRATE_LIM
  Switch Case : SwitchCase  CaseConditions={MotionState.Hold, [MotionState.Brake, MotionState.Move]}  ShowDefaultCase=off
  psi_rate_cmd_radPs : Outport
  wires:
  Move Control/1(psi_rate_cmd_radPs) -> Merge/2
  Hold Control/1(psi_rate_cmd_radPs) -> Merge/1
  In Bus Element/1 -> Hold Control/1(FMS_In)
  Switch Case/2 -> Move Control/Action
  Switch Case/1 -> Hold Control/Action
  motion_state/1 -> Switch Case/1
  Saturation/1 -> psi_rate_cmd_radPs/1
  Merge/1 -> Saturation/1
  In Bus Element1/1 -> Move Control/1(FMS_In)

== system FMS/FMS Commander/Commander/Arm/Assist/Position/Heading Command/Detect Movement ==
  FMS_In : Inport
  Abs : Abs
  Abs1 : Abs
  Bus Selector : BusSelector  OutputSignals=Pilot_Cmd.stick_yaw,INS_Out.r
  Compare To Constant : simulink/Logic and Bit Operations/Compare To Constant  relop=>  const=FMS_PARAM.MC_YAW_DZ  OutDataTypeStr=boolean
  Motion State : Stateflow chart  TreatAsAtomicUnit=on
  motion_state : Outport
  wires:
  FMS_In/1 -> Bus Selector/1
  Abs1/1 -> Compare To Constant/1
  Motion State/1(state) -> motion_state/1
  Compare To Constant/1 -> Motion State/1(motion_req)
  Abs/1 -> Motion State/2(speed)
  Bus Selector/1 -> Abs1/1  "<stick_yaw>"
  Bus Selector/2 -> Abs/1  "<r>"

== system FMS/FMS Commander/Commander/Arm/Assist/Position/Position Command/Controller ==
  motion_state : Inport
  In Bus Element : Inport  Port=2  PortName=FMS_In
  In Bus Element1 : Inport  Port=2  PortName=FMS_In
  Hold Control : Subsystem  TreatAsAtomicUnit=on
  Merge : Merge
  Move Control : Subsystem  TreatAsAtomicUnit=on
  Saturation1 : Saturate  UpperLimit=FMS_PARAM.MC_VEL_XY_LIM  LowerLimit=-FMS_PARAM.MC_VEL_XY_LIM
  Switch Case : SwitchCase  CaseConditions={MotionState.Hold, [MotionState.Brake, MotionState.Move]}  ShowDefaultCase=off
  uv_cmd_mPs : Outport
  wires:
  Move Control/1(uv_cmd_mPs) -> Merge/2
  Hold Control/1(uv_cmd_mPs) -> Merge/1
  In Bus Element/1 -> Hold Control/1(FMS_In)
  Switch Case/2 -> Move Control/Action
  Switch Case/1 -> Hold Control/Action
  motion_state/1 -> Switch Case/1
  Saturation1/1 -> uv_cmd_mPs/1
  Merge/1 -> Saturation1/1
  In Bus Element1/1 -> Move Control/1(FMS_In)

== system FMS/FMS Commander/Commander/Arm/Assist/Position/Position Command/Detect Movement ==
  FMS_In : Inport
  Abs1 : Abs
  Abs2 : Abs
  Add : Sum
  Bus Selector1 : BusSelector  OutputSignals=Pilot_Cmd.stick_pitch,Pilot_Cmd.stick_roll,INS_Out.vn,INS_Out.ve
  Compare To Constant : simulink/Logic and Bit Operations/Compare To Constant  relop=>  const=FMS_PARAM.MC_ROLL_DZ  OutDataTypeStr=boolean
  Compare To Constant1 : simulink/Logic and Bit Operations/Compare To Constant  relop=>  const=FMS_PARAM.MC_PITCH_DZ  OutDataTypeStr=boolean
  Logical Operator : Logic  Operator=OR  AllPortsSameDT=off  OutDataTypeStr=boolean
  Motion State : Stateflow chart  TreatAsAtomicUnit=on
  Sqrt : Sqrt  SaturateOnIntegerOverflow=on
  Square : Math  Operator=square  SaturateOnIntegerOverflow=on
  Square1 : Math  Operator=square  SaturateOnIntegerOverflow=on
  motion_state : Outport
  wires:
  FMS_In/1 -> Bus Selector1/1
  Add/1 -> Sqrt/1
  Square1/1 -> Add/2
  Square/1 -> Add/1
  Logical Operator/1 -> Motion State/1(motion_req)
  Compare To Constant/1 -> Logical Operator/2
  Compare To Constant1/1 -> Logical Operator/1
  Abs2/1 -> Compare To Constant1/1
  Abs1/1 -> Compare To Constant/1
  Motion State/1(state) -> motion_state/1  "pos_ms"
  Sqrt/1 -> Motion State/2(speed)
  Bus Selector1/1 -> Abs2/1  "<stick_pitch>"
  Bus Selector1/2 -> Abs1/1  "<stick_roll>"
  Bus Selector1/3 -> Square/1  "<vn>"
  Bus Selector1/4 -> Square1/1  "<ve>"

== system FMS/FMS Commander/Commander/Arm/Assist/Stabilize/Attitude Command/DeadZone ==
  u : Inport
  Dead Zone : DeadZone  LowerValue=-th  UpperValue=th  SaturateOnIntegerOverflow=on
  Gain : Gain  Gain=1/(1-th)
  y : Outport
  wires:
  Gain/1 -> y/1
  Dead Zone/1 -> Gain/1
  u/1 -> Dead Zone/1

== system FMS/FMS Commander/Commander/Arm/Assist/Stabilize/Attitude Command/DeadZone2 ==
  u : Inport
  Dead Zone : DeadZone  LowerValue=-th  UpperValue=th  SaturateOnIntegerOverflow=on
  Gain : Gain  Gain=1/(1-th)
  y : Outport
  wires:
  u/1 -> Dead Zone/1
  Dead Zone/1 -> Gain/1
  Gain/1 -> y/1

== system FMS/FMS Commander/Commander/Arm/Assist/Stabilize/Attitude Command/Phi_CMD_TD ==
  v : Inport
  Constant : Constant  Value=FMS_PARAM.MC_STICK_SENS
  Integrator : DiscreteIntegrator  SampleTime=-1  ICPrevOutput=DiscIntNeverNeededParam  ICPrevScaledInput=DiscIntNeverNeededParam
  Integrator1 : DiscreteIntegrator  SampleTime=-1  ICPrevOutput=DiscIntNeverNeededParam  ICPrevScaledInput=DiscIntNeverNeededParam
  Subtract : Sum  Inputs=+-
  "fhan " : Subsystem  mask{r0=10*pi, h0=0.04}
      mask DialogControl ParameterGroupVar Prompt: fhan(v1,v2,r0,h0)
  v1 : Outport
  wires:
  "fhan "/1(fhan) -> Integrator/1
  Subtract/1 -> "fhan "/1(v1)
  Integrator/1 -> Integrator1/1, "fhan "/2(v2)  "v2"
  v/1 -> Subtract/2
  Integrator1/1 -> Subtract/1, v1/1
  Constant/1 -> "fhan "/3(scale)

== system FMS/FMS Commander/Commander/Arm/Assist/Stabilize/Attitude Command/Theta_CMD_TD ==
  v : Inport
  Constant : Constant  Value=FMS_PARAM.MC_STICK_SENS
  Integrator : DiscreteIntegrator  SampleTime=-1  ICPrevOutput=DiscIntNeverNeededParam  ICPrevScaledInput=DiscIntNeverNeededParam
  Integrator1 : DiscreteIntegrator  SampleTime=-1  ICPrevOutput=DiscIntNeverNeededParam  ICPrevScaledInput=DiscIntNeverNeededParam
  Subtract : Sum  Inputs=+-
  "fhan " : Subsystem  mask{r0=10*pi, h0=0.04}
      mask DialogControl ParameterGroupVar Prompt: fhan(v1,v2,r0,h0)
  v1 : Outport
  wires:
  Integrator1/1 -> v1/1, Subtract/1
  v/1 -> Subtract/2
  Integrator/1 -> Integrator1/1, "fhan "/2(v2)  "v2"
  Subtract/1 -> "fhan "/1(v1)
  "fhan "/1(fhan) -> Integrator/1
  Constant/1 -> "fhan "/3(scale)
